simulink model "Pole_placement_simulation_DT"  (R2023b)
settings: Solver=VariableStepAuto  StartTime=0.0  StopTime=15  RelTol=1e-3
values from neighbouring files (symbols this model uses):
  A = [0 1 0 0;32.79 0 6.625 0;0 0 0 1;-67.38 0 -8.92 0]    [Pole_placement_DT.m]
  B = [0 0; 4.65 -7.94;0 0;-7.94 27.27]    [Pole_placement_DT.m]
  gainMatrix = dcgain(transferFunctionPos^-1)    [Pole_placement_DT.m]
  K = place(Ad,Bd,zcc)    [Pole_placement_DT.m]
  Kfinal = place(Adaug,Bdaug,zcci)    [Pole_placement_DT.m]
  Ts = 0.1    [Pole_placement_DT.m]
undefined symbols (not defined in the file or in its folder): Ad, Bd, Cd, Dd, DiscIntNeverNeededParam
settings Model: Creator=Giammo  LastModifiedBy=Giammo

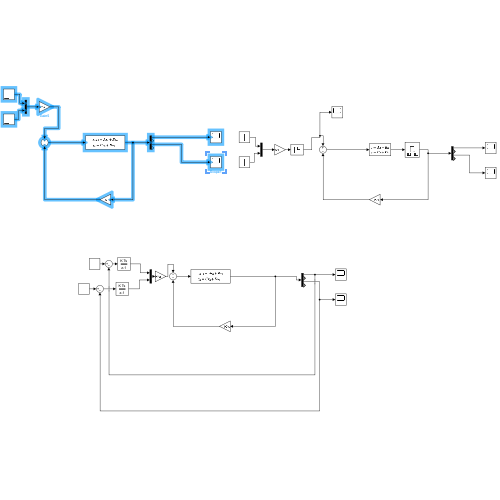
[thumbnail: Simulink's stored preview of the top-level diagram]
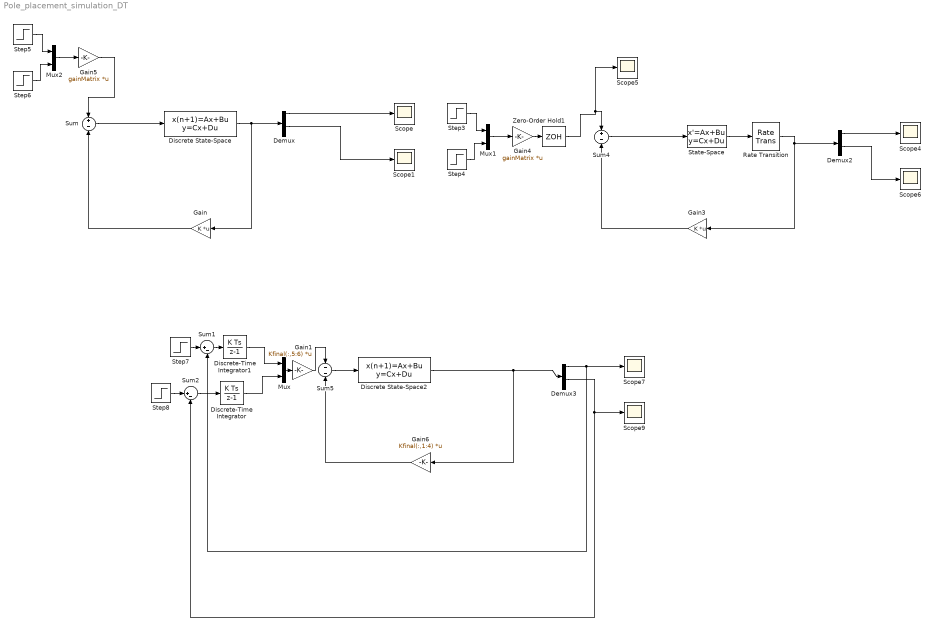
== system Pole_placement_simulation_DT ==
  Demux : Demux
  Demux2 : Demux
  Demux3 : Demux
  Discrete State-Space : DiscreteStateSpace  A=Ad  B=Bd  C=Cd  D=Dd  SampleTime=Ts
  Discrete State-Space2 : DiscreteStateSpace  A=Ad  B=Bd  C=Cd  D=Dd  SampleTime=Ts
  Discrete-Time Integrator : DiscreteIntegrator  SampleTime=Ts  ICPrevOutput=DiscIntNeverNeededParam  ICPrevScaledInput=DiscIntNeverNeededParam
  Discrete-Time Integrator1 : DiscreteIntegrator  SampleTime=Ts  ICPrevOutput=DiscIntNeverNeededParam  ICPrevScaledInput=DiscIntNeverNeededParam
  Gain : Gain  Gain=K  Multiplication=Matrix(K*u)
  Gain1 : Gain  Gain=Kfinal(:,5:6)  Multiplication=Matrix(K*u)
  Gain3 : Gain  Gain=K  Multiplication=Matrix(K*u)
  Gain4 : Gain  Gain=gainMatrix  Multiplication=Matrix(K*u)
  Gain5 : Gain  Gain=gainMatrix  Multiplication=Matrix(K*u)
  Gain6 : Gain  Gain=Kfinal(:,1:4)  Multiplication=Matrix(K*u)
  Mux : Mux  Inputs=2
  Mux1 : Mux  Inputs=2
  Mux2 : Mux  Inputs=2
  Rate Transition : RateTransition  OutPortSampleTime=Ts
  Scope{,1,4..7,9} (7 alike) : Scope
  State-Space : StateSpace  A=A  B=B  C=eye(4)  D=zeros(4,2)  InitialCondition=0
  Step{3..8} (6 alike) : Step  After=0.26  SampleTime=0
  Sum : Sum  Inputs=+-
  Sum1 : Sum  Inputs=|+-
  Sum2 : Sum  Inputs=|+-
  Sum4 : Sum  Inputs=+-
  Sum5 : Sum  Inputs=--
  Zero-Order Hold1 : ZeroOrderHold  SampleTime=Ts
  wires:
  Discrete State-Space/1 -> Gain/1, Demux/1
  Gain/1 -> Sum/2
  Demux/1 -> Scope/1
  Sum/1 -> Discrete State-Space/1
  Demux/3 -> Scope1/1
  Rate Transition/1 -> Gain3/1, Demux2/1
  Zero-Order Hold1/1 -> Scope5/1, Sum4/1
  Gain3/1 -> Sum4/2
  Sum4/1 -> State-Space/1
  Demux2/1 -> Scope4/1
  Demux2/3 -> Scope6/1
  Gain4/1 -> Zero-Order Hold1/1
  Step3/1 -> Mux1/1
  Step4/1 -> Mux1/2
  Mux1/1 -> Gain4/1
  Gain5/1 -> Sum/1
  Step6/1 -> Mux2/2
  Step5/1 -> Mux2/1
  Mux2/1 -> Gain5/1
  Gain6/1 -> Sum5/2
  Step7/1 -> Sum1/1
  Sum1/1 -> Discrete-Time Integrator1/1
  Demux3/1 -> Scope7/1, Sum1/2
  State-Space/1 -> Rate Transition/1
  Step8/1 -> Sum2/1
  Sum2/1 -> Discrete-Time Integrator/1
  Demux3/3 -> Sum2/2, Scope9/1
  Discrete-Time Integrator1/1 -> Mux/1
  Discrete-Time Integrator/1 -> Mux/2
  Sum5/1 -> Discrete State-Space2/1
  Discrete State-Space2/1 -> Gain6/1, Demux3/1
  Mux/1 -> Gain1/1
  Gain1/1 -> Sum5/1
